simulink model "GetSetParamExample"  (R2023b)
settings: Solver=ode45  StartTime=0.0  StopTime=7e-2  MaxStep=1e-4  RelTol=1e-3
libraries: simulink x2
settings Model: Creator=rlschie  LastModifiedBy=rlschie

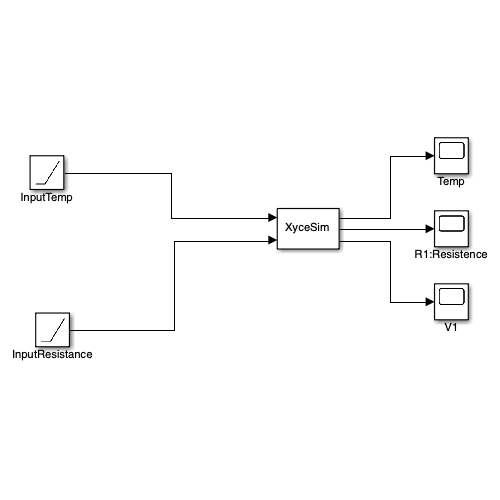
[thumbnail: Simulink's stored preview of the top-level diagram]
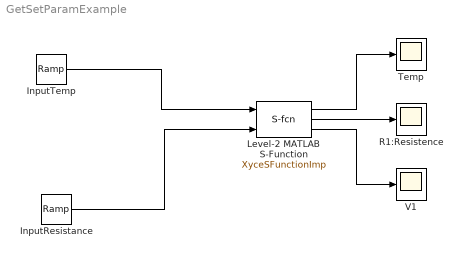
== system GetSetParamExample ==
  InputResistance : simulink/Sources/Ramp  slope=500  start=0  InitialOutput=100
  InputTemp : simulink/Sources/Ramp  slope=-50  start=1e-3  InitialOutput=20
  Level-2 MATLAB S-Function : M-S-Function  FunctionName=XyceSFunctionImp  Parameters=XyceInputFileName,WorkingDirectory,NumberOfInputs,NumberOfOutputs,InputNames,OutputNames  mask{XyceInputFileName=GetSetParams.cir, WorkingDirectory=/Users/rlschie/src/XyceDevelopment/Xyce/utils/SimulinkInterface/SimulinkExamples/, XyceInputPortNames=, XyceOutputPortNames=, XyceNumberOfInputPorts=0, XyceNumberOfOutputPorts=0, NumberOfInputs=2, NumberOfOutputs=3, InputNames={ '1', 'TEMP'; '2', 'R1:R' }, OutputNames={ '1', 'TEMP'; '2', 'R1:R'; '3', 'V(1)' }}
      mask prompts: XyceInputFileName "Xyce Input Filename"; WorkingDirectory "Working Directory"; XyceInputPortNames "Xyce Input Port Names"; XyceOutputPortNames "Xyce Output Port Names"; XyceNumberOfInputPorts "Xyce Number Of Inputs"; XyceNumberOfOutputPorts "Xyce Number Of Outputs"; NumberOfInputs "Number of Inputs"; NumberOfOutputs "Number of Outputs"; InputNames "Input Names"; OutputNames "Output Names"
      mask DialogControl SelectXyceInputFileButton Prompt: Select Xyce Input File
      mask DialogControl ScanXyceInputFileButton Prompt: Scan Xyce Input File
      mask DialogControl ResetForm Prompt: Reset
      mask DialogControl AddInputLineButton Prompt: Add Line
      mask DialogControl RemoveInputLineButton Prompt: Remove Line
      mask DialogControl AddOutputLineButton Prompt: Add Line
      mask DialogControl RemoveOutputLineButton Prompt: Remove Line
      mask Display: disp('XyceSim');
  R1:Resistence : Scope
  Temp : Scope
  V1 : Scope
  wires:
  InputTemp/1 -> Level-2 MATLAB S-Function/1
  InputResistance/1 -> Level-2 MATLAB S-Function/2
  Level-2 MATLAB S-Function/1 -> Temp/1
  Level-2 MATLAB S-Function/2 -> R1:Resistence/1
  Level-2 MATLAB S-Function/3 -> V1/1
